simulink model "fault_detection_system_v8"  (R2024a)
settings: Solver=FixedStepDiscrete  StartTime=0.0  StopTime=2  FixedStep=1e-4  RelTol=1e-3
settings Model: Creator=UJJWAL  LastModifiedBy=UJJWAL

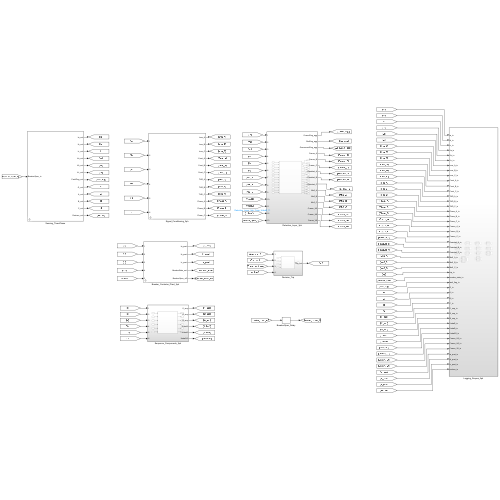
[thumbnail: Simulink's stored preview of the top-level diagram]
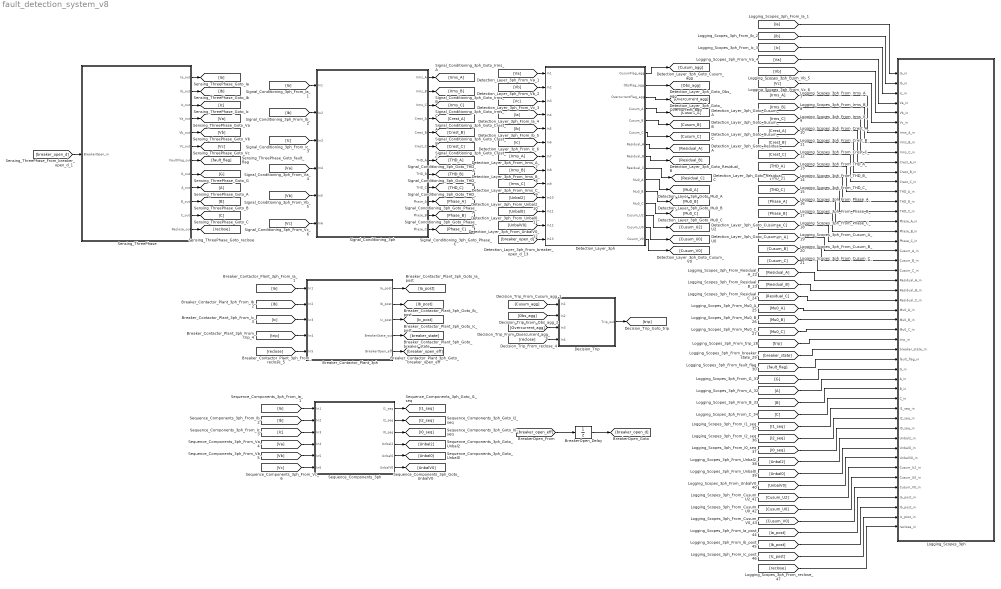
== system fault_detection_system_v8 ==
  BreakerOpen_Delay : UnitDelay  SampleTime=1e-4  HasFrameUpgradeWarning=on
  Breaker_Contactor_Plant_3ph : Subsystem  mask{FeedbackEnable=0, BreakerDelay=0.040000}
      mask prompts: FeedbackEnable "Feedback enable (1 = breaker interrupts the plant, 0 = latch only)"; BreakerDelay "Breaker opening delay after trip command (s)"
  Decision_Trip : Subsystem
  Detection_Layer_3ph : Subsystem
  Logging_Scopes_3ph : Subsystem
  Logging_Scopes_3ph_From_A_32 : From
  Sensing_ThreePhase : Subsystem  mask{FaultG=off, FaultA=on, FaultB=on, FaultC=on, MechanismCode=6, Severity=2750, RampDuration=0, FaultOnsetTime=0.400000, FaultDuration=1.000000, SourceL=0.005, ReclosDelay=0.100000}
      mask prompts: FaultG "Ground involved (G)"; FaultA "Phase A involved"; FaultB "Phase B involved"; FaultC "Phase C involved"; MechanismCode "Mechanism code"; RampDuration "Ramp duration (s)"; FaultOnsetTime "Fault onset time (s)"; FaultDuration "Fault duration (s)"; SourceL "Source inductance (H), 0 = v6 behaviour"; ReclosDelay "Reclose delay after clearance (s)"
  Sensing_ThreePhase_Goto_A : Goto
  Sequence_Components_3ph : Subsystem
  Signal_Conditioning_3ph : Subsystem  mask{NoiseSeed=3028}
      mask prompts: NoiseSeed "Noise seed"
  wires:
  Sensing_ThreePhase/1(Ia_out) -> [Ia]
  Sensing_ThreePhase/2(Ib_out) -> [Ib]
  Sensing_ThreePhase/3(Ic_out) -> [Ic]
  Sensing_ThreePhase/4(Va_out) -> [Va]
  Sensing_ThreePhase/5(Vb_out) -> [Vb]
  Sensing_ThreePhase/6(Vc_out) -> [Vc]
  Sensing_ThreePhase/7(FaultFlag_out) -> [fault_flag]
  Sensing_ThreePhase/8(G_out) -> [G]
  Sensing_ThreePhase/9(A_out) -> Sensing_ThreePhase_Goto_A/1
  Sensing_ThreePhase/10(B_out) -> [B]
  Sensing_ThreePhase/11(C_out) -> [C]
  Sensing_ThreePhase/12(Reclose_out) -> [reclose]
  Signal_Conditioning_3ph/1(Irms_A) -> [Irms_A]
  Signal_Conditioning_3ph/2(Irms_B) -> [Irms_B]
  Signal_Conditioning_3ph/3(Irms_C) -> [Irms_C]
  Signal_Conditioning_3ph/4(Crest_A) -> [Crest_A]
  Signal_Conditioning_3ph/5(Crest_B) -> [Crest_B]
  Signal_Conditioning_3ph/6(Crest_C) -> [Crest_C]
  Signal_Conditioning_3ph/7(THD_A) -> [THD_A]
  Signal_Conditioning_3ph/8(THD_B) -> [THD_B]
  Signal_Conditioning_3ph/9(THD_C) -> [THD_C]
  Signal_Conditioning_3ph/10(Phase_A) -> [Phase_A]
  Signal_Conditioning_3ph/11(Phase_B) -> [Phase_B]
  Signal_Conditioning_3ph/12(Phase_C) -> [Phase_C]
  Sequence_Components_3ph/1(I1_seq) -> [I1_seq]
  Sequence_Components_3ph/2(I2_seq) -> [I2_seq]
  Sequence_Components_3ph/3(I0_seq) -> [I0_seq]
  Sequence_Components_3ph/4(Unbal2) -> [Unbal2]
  Sequence_Components_3ph/5(Unbal0) -> [Unbal0]
  Sequence_Components_3ph/6(UnbalV0) -> [UnbalV0]
  Detection_Layer_3ph/1(CusumFlag_agg) -> [Cusum_agg]
  Detection_Layer_3ph/2(ObsFlag_agg) -> [Obs_agg]
  Detection_Layer_3ph/3(OvercurrentFlag_agg) -> [Overcurrent_agg]
  Detection_Layer_3ph/4(Cusum_A) -> [Cusum_A]
  Detection_Layer_3ph/5(Cusum_B) -> [Cusum_B]
  Detection_Layer_3ph/6(Cusum_C) -> [Cusum_C]
  Detection_Layer_3ph/7(Residual_A) -> [Residual_A]
  Detection_Layer_3ph/8(Residual_B) -> [Residual_B]
  Detection_Layer_3ph/9(Residual_C) -> [Residual_C]
  Detection_Layer_3ph/10(Mu0_A) -> [Mu0_A]
  Detection_Layer_3ph/11(Mu0_B) -> [Mu0_B]
  Detection_Layer_3ph/12(Mu0_C) -> [Mu0_C]
  Detection_Layer_3ph/13(Cusum_U2) -> [Cusum_U2]
  Detection_Layer_3ph/14(Cusum_U0) -> [Cusum_U0]
  Detection_Layer_3ph/15(Cusum_V0) -> [Cusum_V0]
  Decision_Trip/1(Trip_out) -> [trip]
  Breaker_Contactor_Plant_3ph/1(Ia_post) -> [Ia_post]
  Breaker_Contactor_Plant_3ph/2(Ib_post) -> [Ib_post]
  Breaker_Contactor_Plant_3ph/3(Ic_post) -> [Ic_post]
  Breaker_Contactor_Plant_3ph/4(BreakerState_out) -> [breaker_state]
  Breaker_Contactor_Plant_3ph/5(BreakerOpen_eff) -> [breaker_open_eff]
  [breaker_open_d] -> Sensing_ThreePhase/1(BreakerOpen_in)
  [Ia] -> Signal_Conditioning_3ph/1(In1)
  [Ib] -> Signal_Conditioning_3ph/2(In2)
  [Ic] -> Signal_Conditioning_3ph/3(In3)
  [Va] -> Signal_Conditioning_3ph/4(In4)
  [Vb] -> Signal_Conditioning_3ph/5(In5)
  [Vc] -> Signal_Conditioning_3ph/6(In6)
  [Ia] -> Sequence_Components_3ph/1(In1)
  [Ib] -> Sequence_Components_3ph/2(In2)
  [Ic] -> Sequence_Components_3ph/3(In3)
  [Va] -> Sequence_Components_3ph/4(In4)
  [Vb] -> Sequence_Components_3ph/5(In5)
  [Vc] -> Sequence_Components_3ph/6(In6)
  [Va] -> Detection_Layer_3ph/1(In1)
  [Vb] -> Detection_Layer_3ph/2(In2)
  [Vc] -> Detection_Layer_3ph/3(In3)
  [Ia] -> Detection_Layer_3ph/4(In4)
  [Ib] -> Detection_Layer_3ph/5(In5)
  [Ic] -> Detection_Layer_3ph/6(In6)
  [Irms_A] -> Detection_Layer_3ph/7(In7)
  [Irms_B] -> Detection_Layer_3ph/8(In8)
  [Irms_C] -> Detection_Layer_3ph/9(In9)
  [Unbal2] -> Detection_Layer_3ph/10(In10)
  [Unbal0] -> Detection_Layer_3ph/11(In11)
  [UnbalV0] -> Detection_Layer_3ph/12(In12)
  [breaker_open_d] -> Detection_Layer_3ph/13(In13)
  [Cusum_agg] -> Decision_Trip/1(In1)
  [Obs_agg] -> Decision_Trip/2(In2)
  [Overcurrent_agg] -> Decision_Trip/3(In3)
  [reclose] -> Decision_Trip/4(In4)
  [Ia] -> Breaker_Contactor_Plant_3ph/1(In1)
  [Ib] -> Breaker_Contactor_Plant_3ph/2(In2)
  [Ic] -> Breaker_Contactor_Plant_3ph/3(In3)
  [trip] -> Breaker_Contactor_Plant_3ph/4(In4)
  [reclose] -> Breaker_Contactor_Plant_3ph/5(In5)
  [Ia] -> Logging_Scopes_3ph/1(Ia_in)
  [Ib] -> Logging_Scopes_3ph/2(Ib_in)
  [Ic] -> Logging_Scopes_3ph/3(Ic_in)
  [Va] -> Logging_Scopes_3ph/4(Va_in)
  [Vb] -> Logging_Scopes_3ph/5(Vb_in)
  [Vc] -> Logging_Scopes_3ph/6(Vc_in)
  [Irms_A] -> Logging_Scopes_3ph/7(Irms_A_in)
  [Irms_B] -> Logging_Scopes_3ph/8(Irms_B_in)
  [Irms_C] -> Logging_Scopes_3ph/9(Irms_C_in)
  [Crest_A] -> Logging_Scopes_3ph/10(Crest_A_in)
  [Crest_B] -> Logging_Scopes_3ph/11(Crest_B_in)
  [Crest_C] -> Logging_Scopes_3ph/12(Crest_C_in)
  [THD_A] -> Logging_Scopes_3ph/13(THD_A_in)
  [THD_B] -> Logging_Scopes_3ph/14(THD_B_in)
  [THD_C] -> Logging_Scopes_3ph/15(THD_C_in)
  [Phase_A] -> Logging_Scopes_3ph/16(Phase_A_in)
  [Phase_B] -> Logging_Scopes_3ph/17(Phase_B_in)
  [Phase_C] -> Logging_Scopes_3ph/18(Phase_C_in)
  [Cusum_A] -> Logging_Scopes_3ph/19(Cusum_A_in)
  [Cusum_B] -> Logging_Scopes_3ph/20(Cusum_B_in)
  [Cusum_C] -> Logging_Scopes_3ph/21(Cusum_C_in)
  [Residual_A] -> Logging_Scopes_3ph/22(Residual_A_in)
  [Residual_B] -> Logging_Scopes_3ph/23(Residual_B_in)
  [Residual_C] -> Logging_Scopes_3ph/24(Residual_C_in)
  [Mu0_A] -> Logging_Scopes_3ph/25(Mu0_A_in)
  [Mu0_B] -> Logging_Scopes_3ph/26(Mu0_B_in)
  [Mu0_C] -> Logging_Scopes_3ph/27(Mu0_C_in)
  [trip] -> Logging_Scopes_3ph/28(trip_in)
  [breaker_state] -> Logging_Scopes_3ph/29(breaker_state_in)
  [fault_flag] -> Logging_Scopes_3ph/30(fault_flag_in)
  [G] -> Logging_Scopes_3ph/31(G_in)
  Logging_Scopes_3ph_From_A_32/1 -> Logging_Scopes_3ph/32(A_in)
  [B] -> Logging_Scopes_3ph/33(B_in)
  [C] -> Logging_Scopes_3ph/34(C_in)
  [I1_seq] -> Logging_Scopes_3ph/35(I1_seq_in)
  [I2_seq] -> Logging_Scopes_3ph/36(I2_seq_in)
  [I0_seq] -> Logging_Scopes_3ph/37(I0_seq_in)
  [Unbal2] -> Logging_Scopes_3ph/38(Unbal2_in)
  [Unbal0] -> Logging_Scopes_3ph/39(Unbal0_in)
  [UnbalV0] -> Logging_Scopes_3ph/40(UnbalV0_in)
  [Cusum_U2] -> Logging_Scopes_3ph/41(Cusum_U2_in)
  [Cusum_U0] -> Logging_Scopes_3ph/42(Cusum_U0_in)
  [Cusum_V0] -> Logging_Scopes_3ph/43(Cusum_V0_in)
  [Ia_post] -> Logging_Scopes_3ph/44(Ia_post_in)
  [Ib_post] -> Logging_Scopes_3ph/45(Ib_post_in)
  [Ic_post] -> Logging_Scopes_3ph/46(Ic_post_in)
  [reclose] -> Logging_Scopes_3ph/47(reclose_in)
  [breaker_open_eff] -> BreakerOpen_Delay/1
  BreakerOpen_Delay/1 -> [breaker_open_d]

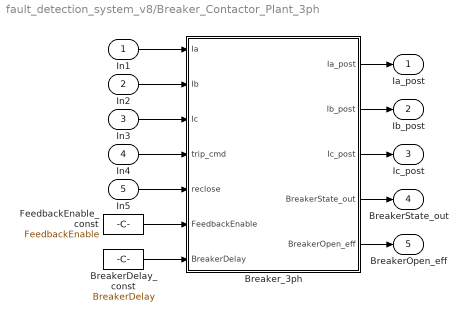
== system fault_detection_system_v8/Breaker_Contactor_Plant_3ph ==
  In1 : Inport
  In2 : Inport  Port=2
  In3 : Inport  Port=3
  In4 : Inport  Port=4
  In5 : Inport  Port=5
  BreakerDelay_const : Constant  Value=BreakerDelay
  Breaker_3ph : MATLAB Function  TreatAsAtomicUnit=on
  FeedbackEnable_const : Constant  Value=FeedbackEnable
  Ia_post : Outport
  Ib_post : Outport  Port=2
  Ic_post : Outport  Port=3
  BreakerState_out : Outport  Port=4
  BreakerOpen_eff : Outport  Port=5
  wires:
  Breaker_3ph/1(Ia_post) -> Ia_post/1
  Breaker_3ph/2(Ib_post) -> Ib_post/1
  Breaker_3ph/3(Ic_post) -> Ic_post/1
  Breaker_3ph/4(BreakerState_out) -> BreakerState_out/1
  Breaker_3ph/5(BreakerOpen_eff) -> BreakerOpen_eff/1
  In1/1 -> Breaker_3ph/1(Ia)
  In2/1 -> Breaker_3ph/2(Ib)
  In3/1 -> Breaker_3ph/3(Ic)
  In4/1 -> Breaker_3ph/4(trip_cmd)
  In5/1 -> Breaker_3ph/5(reclose)
  FeedbackEnable_const/1 -> Breaker_3ph/6(FeedbackEnable)
  BreakerDelay_const/1 -> Breaker_3ph/7(BreakerDelay)

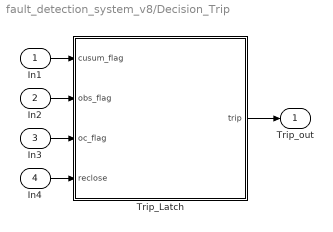
== system fault_detection_system_v8/Decision_Trip ==
  In1 : Inport
  In2 : Inport  Port=2
  In3 : Inport  Port=3
  In4 : Inport  Port=4
  Trip_Latch : MATLAB Function  TreatAsAtomicUnit=on
  Trip_out : Outport
  wires:
  In1/1 -> Trip_Latch/1(cusum_flag)
  In2/1 -> Trip_Latch/2(obs_flag)
  In3/1 -> Trip_Latch/3(oc_flag)
  In4/1 -> Trip_Latch/4(reclose)
  Trip_Latch/1(trip) -> Trip_out/1

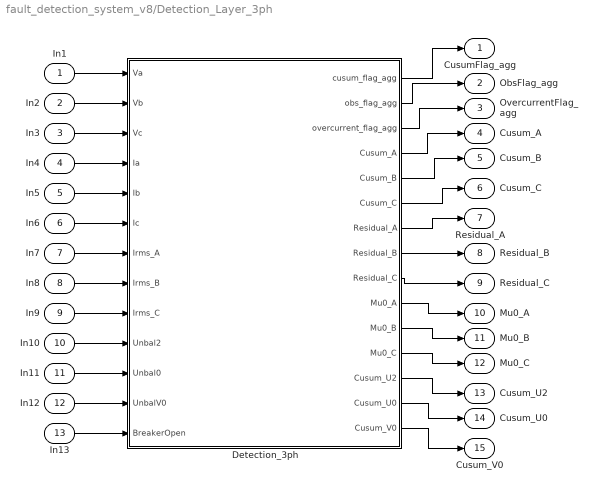
== system fault_detection_system_v8/Detection_Layer_3ph ==
  In1 : Inport
  In2 : Inport  Port=2
  In3 : Inport  Port=3
  In4 : Inport  Port=4
  In5 : Inport  Port=5
  In6 : Inport  Port=6
  In7 : Inport  Port=7
  In8 : Inport  Port=8
  In9 : Inport  Port=9
  In10 : Inport  Port=10
  In11 : Inport  Port=11
  In12 : Inport  Port=12
  In13 : Inport  Port=13
  Detection_3ph : MATLAB Function  TreatAsAtomicUnit=on
  CusumFlag_agg : Outport
  ObsFlag_agg : Outport  Port=2
  OvercurrentFlag_agg : Outport  Port=3
  Cusum_A : Outport  Port=4
  Cusum_B : Outport  Port=5
  Cusum_C : Outport  Port=6
  Residual_A : Outport  Port=7
  Residual_B : Outport  Port=8
  Residual_C : Outport  Port=9
  Mu0_A : Outport  Port=10
  Mu0_B : Outport  Port=11
  Mu0_C : Outport  Port=12
  Cusum_U2 : Outport  Port=13
  Cusum_U0 : Outport  Port=14
  Cusum_V0 : Outport  Port=15
  wires:
  Detection_3ph/1(cusum_flag_agg) -> CusumFlag_agg/1
  Detection_3ph/2(obs_flag_agg) -> ObsFlag_agg/1
  Detection_3ph/3(overcurrent_flag_agg) -> OvercurrentFlag_agg/1
  Detection_3ph/4(Cusum_A) -> Cusum_A/1
  Detection_3ph/5(Cusum_B) -> Cusum_B/1
  Detection_3ph/6(Cusum_C) -> Cusum_C/1
  Detection_3ph/7(Residual_A) -> Residual_A/1
  Detection_3ph/8(Residual_B) -> Residual_B/1
  Detection_3ph/9(Residual_C) -> Residual_C/1
  Detection_3ph/10(Mu0_A) -> Mu0_A/1
  Detection_3ph/11(Mu0_B) -> Mu0_B/1
  Detection_3ph/12(Mu0_C) -> Mu0_C/1
  Detection_3ph/13(Cusum_U2) -> Cusum_U2/1
  Detection_3ph/14(Cusum_U0) -> Cusum_U0/1
  Detection_3ph/15(Cusum_V0) -> Cusum_V0/1
  In1/1 -> Detection_3ph/1(Va)
  In2/1 -> Detection_3ph/2(Vb)
  In3/1 -> Detection_3ph/3(Vc)
  In4/1 -> Detection_3ph/4(Ia)
  In5/1 -> Detection_3ph/5(Ib)
  In6/1 -> Detection_3ph/6(Ic)
  In7/1 -> Detection_3ph/7(Irms_A)
  In8/1 -> Detection_3ph/8(Irms_B)
  In9/1 -> Detection_3ph/9(Irms_C)
  In10/1 -> Detection_3ph/10(Unbal2)
  In11/1 -> Detection_3ph/11(Unbal0)
  In12/1 -> Detection_3ph/12(UnbalV0)
  In13/1 -> Detection_3ph/13(BreakerOpen)

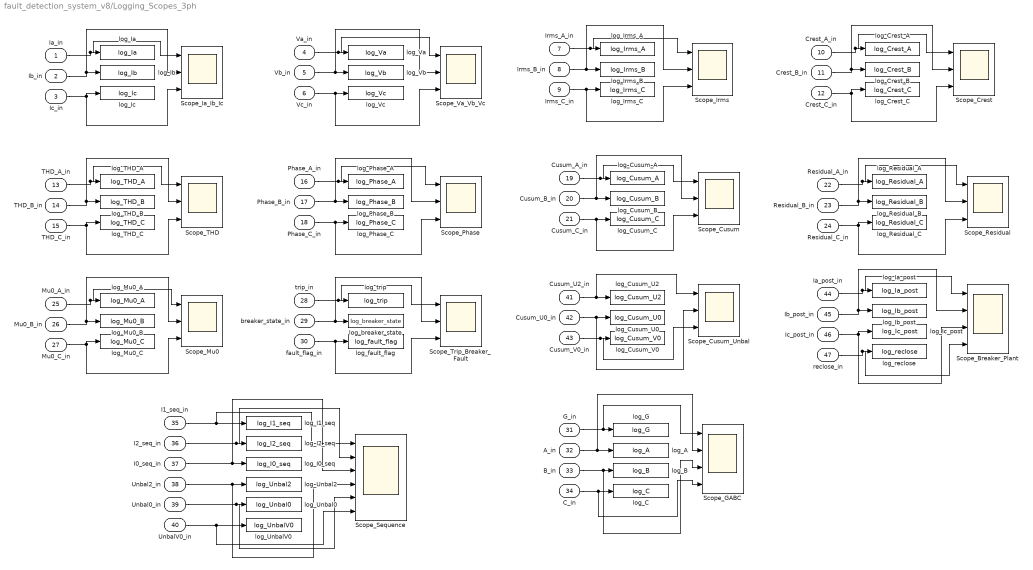
== system fault_detection_system_v8/Logging_Scopes_3ph ==
  Ia_in : Inport
  Ib_in : Inport  Port=2
  Ic_in : Inport  Port=3
  Va_in : Inport  Port=4
  Vb_in : Inport  Port=5
  Vc_in : Inport  Port=6
  Irms_A_in : Inport  Port=7
  Irms_B_in : Inport  Port=8
  Irms_C_in : Inport  Port=9
  Crest_A_in : Inport  Port=10
  Crest_B_in : Inport  Port=11
  Crest_C_in : Inport  Port=12
  THD_A_in : Inport  Port=13
  THD_B_in : Inport  Port=14
  THD_C_in : Inport  Port=15
  Phase_A_in : Inport  Port=16
  Phase_B_in : Inport  Port=17
  Phase_C_in : Inport  Port=18
  Cusum_A_in : Inport  Port=19
  Cusum_B_in : Inport  Port=20
  Cusum_C_in : Inport  Port=21
  Residual_A_in : Inport  Port=22
  Residual_B_in : Inport  Port=23
  Residual_C_in : Inport  Port=24
  Mu0_A_in : Inport  Port=25
  Mu0_B_in : Inport  Port=26
  Mu0_C_in : Inport  Port=27
  trip_in : Inport  Port=28
  breaker_state_in : Inport  Port=29
  fault_flag_in : Inport  Port=30
  G_in : Inport  Port=31
  A_in : Inport  Port=32
  B_in : Inport  Port=33
  C_in : Inport  Port=34
  I1_seq_in : Inport  Port=35
  I2_seq_in : Inport  Port=36
  I0_seq_in : Inport  Port=37
  Unbal2_in : Inport  Port=38
  Unbal0_in : Inport  Port=39
  UnbalV0_in : Inport  Port=40
  Cusum_U2_in : Inport  Port=41
  Cusum_U0_in : Inport  Port=42
  Cusum_V0_in : Inport  Port=43
  Ia_post_in : Inport  Port=44
  Ib_post_in : Inport  Port=45
  Ic_post_in : Inport  Port=46
  reclose_in : Inport  Port=47
  Scope_Breaker_Plant : Scope  NumInputPorts=4
  Scope_Crest : Scope  NumInputPorts=3
  Scope_Cusum : Scope  NumInputPorts=3
  Scope_Cusum_Unbal : Scope  NumInputPorts=3
  Scope_GABC : Scope  NumInputPorts=4
  Scope_Ia_Ib_Ic : Scope  NumInputPorts=3
  Scope_Irms : Scope  NumInputPorts=3
  Scope_Mu0 : Scope  NumInputPorts=3
  Scope_Phase : Scope  NumInputPorts=3
  Scope_Residual : Scope  NumInputPorts=3
  Scope_Sequence : Scope  NumInputPorts=6
  Scope_THD : Scope  NumInputPorts=3
  Scope_Trip_Breaker_Fault : Scope  NumInputPorts=3
  Scope_Va_Vb_Vc : Scope  NumInputPorts=3
  log_A : ToWorkspace  VariableName=log_A  SaveFormat=Timeseries  SampleTime=-1
  log_B : ToWorkspace  VariableName=log_B  SaveFormat=Timeseries  SampleTime=-1
  log_C : ToWorkspace  VariableName=log_C  SaveFormat=Timeseries  SampleTime=-1
  log_Crest_A : ToWorkspace  VariableName=log_Crest_A  SaveFormat=Timeseries  SampleTime=-1
  log_Crest_B : ToWorkspace  VariableName=log_Crest_B  SaveFormat=Timeseries  SampleTime=-1
  log_Crest_C : ToWorkspace  VariableName=log_Crest_C  SaveFormat=Timeseries  SampleTime=-1
  log_Cusum_A : ToWorkspace  VariableName=log_Cusum_A  SaveFormat=Timeseries  SampleTime=-1
  log_Cusum_B : ToWorkspace  VariableName=log_Cusum_B  SaveFormat=Timeseries  SampleTime=-1
  log_Cusum_C : ToWorkspace  VariableName=log_Cusum_C  SaveFormat=Timeseries  SampleTime=-1
  log_Cusum_U0 : ToWorkspace  VariableName=log_Cusum_U0  SaveFormat=Timeseries  SampleTime=-1
  log_Cusum_U2 : ToWorkspace  VariableName=log_Cusum_U2  SaveFormat=Timeseries  SampleTime=-1
  log_Cusum_V0 : ToWorkspace  VariableName=log_Cusum_V0  SaveFormat=Timeseries  SampleTime=-1
  log_G : ToWorkspace  VariableName=log_G  SaveFormat=Timeseries  SampleTime=-1
  log_I0_seq : ToWorkspace  VariableName=log_I0_seq  SaveFormat=Timeseries  SampleTime=-1
  log_I1_seq : ToWorkspace  VariableName=log_I1_seq  SaveFormat=Timeseries  SampleTime=-1
  log_I2_seq : ToWorkspace  VariableName=log_I2_seq  SaveFormat=Timeseries  SampleTime=-1
  log_Ia : ToWorkspace  VariableName=log_Ia  SaveFormat=Timeseries  SampleTime=-1
  log_Ia_post : ToWorkspace  VariableName=log_Ia_post  SaveFormat=Timeseries  SampleTime=-1
  log_Ib : ToWorkspace  VariableName=log_Ib  SaveFormat=Timeseries  SampleTime=-1
  log_Ib_post : ToWorkspace  VariableName=log_Ib_post  SaveFormat=Timeseries  SampleTime=-1
  log_Ic : ToWorkspace  VariableName=log_Ic  SaveFormat=Timeseries  SampleTime=-1
  log_Ic_post : ToWorkspace  VariableName=log_Ic_post  SaveFormat=Timeseries  SampleTime=-1
  log_Irms_A : ToWorkspace  VariableName=log_Irms_A  SaveFormat=Timeseries  SampleTime=-1
  log_Irms_B : ToWorkspace  VariableName=log_Irms_B  SaveFormat=Timeseries  SampleTime=-1
  log_Irms_C : ToWorkspace  VariableName=log_Irms_C  SaveFormat=Timeseries  SampleTime=-1
  log_Mu0_A : ToWorkspace  VariableName=log_Mu0_A  SaveFormat=Timeseries  SampleTime=-1
  log_Mu0_B : ToWorkspace  VariableName=log_Mu0_B  SaveFormat=Timeseries  SampleTime=-1
  log_Mu0_C : ToWorkspace  VariableName=log_Mu0_C  SaveFormat=Timeseries  SampleTime=-1
  log_Phase_A : ToWorkspace  VariableName=log_Phase_A  SaveFormat=Timeseries  SampleTime=-1
  log_Phase_B : ToWorkspace  VariableName=log_Phase_B  SaveFormat=Timeseries  SampleTime=-1
  log_Phase_C : ToWorkspace  VariableName=log_Phase_C  SaveFormat=Timeseries  SampleTime=-1
  log_Residual_A : ToWorkspace  VariableName=log_Residual_A  SaveFormat=Timeseries  SampleTime=-1
  log_Residual_B : ToWorkspace  VariableName=log_Residual_B  SaveFormat=Timeseries  SampleTime=-1
  log_Residual_C : ToWorkspace  VariableName=log_Residual_C  SaveFormat=Timeseries  SampleTime=-1
  log_THD_A : ToWorkspace  VariableName=log_THD_A  SaveFormat=Timeseries  SampleTime=-1
  log_THD_B : ToWorkspace  VariableName=log_THD_B  SaveFormat=Timeseries  SampleTime=-1
  log_THD_C : ToWorkspace  VariableName=log_THD_C  SaveFormat=Timeseries  SampleTime=-1
  log_Unbal0 : ToWorkspace  VariableName=log_Unbal0  SaveFormat=Timeseries  SampleTime=-1
  log_Unbal2 : ToWorkspace  VariableName=log_Unbal2  SaveFormat=Timeseries  SampleTime=-1
  log_UnbalV0 : ToWorkspace  VariableName=log_UnbalV0  SaveFormat=Timeseries  SampleTime=-1
  log_Va : ToWorkspace  VariableName=log_Va  SaveFormat=Timeseries  SampleTime=-1
  log_Vb : ToWorkspace  VariableName=log_Vb  SaveFormat=Timeseries  SampleTime=-1
  log_Vc : ToWorkspace  VariableName=log_Vc  SaveFormat=Timeseries  SampleTime=-1
  log_breaker_state : ToWorkspace  VariableName=log_breaker_state  SaveFormat=Timeseries  SampleTime=-1
  log_fault_flag : ToWorkspace  VariableName=log_fault_flag  SaveFormat=Timeseries  SampleTime=-1
  log_reclose : ToWorkspace  VariableName=log_reclose  SaveFormat=Timeseries  SampleTime=-1
  log_trip : ToWorkspace  VariableName=log_trip  SaveFormat=Timeseries  SampleTime=-1
  wires:
  Ia_in/1 -> log_Ia/1, Scope_Ia_Ib_Ic/1
  Ib_in/1 -> log_Ib/1, Scope_Ia_Ib_Ic/2
  Ic_in/1 -> log_Ic/1, Scope_Ia_Ib_Ic/3
  Va_in/1 -> log_Va/1, Scope_Va_Vb_Vc/1
  Vb_in/1 -> log_Vb/1, Scope_Va_Vb_Vc/2
  Vc_in/1 -> log_Vc/1, Scope_Va_Vb_Vc/3
  Irms_A_in/1 -> log_Irms_A/1, Scope_Irms/1
  Irms_B_in/1 -> log_Irms_B/1, Scope_Irms/2
  Irms_C_in/1 -> log_Irms_C/1, Scope_Irms/3
  Crest_A_in/1 -> log_Crest_A/1, Scope_Crest/1
  Crest_B_in/1 -> log_Crest_B/1, Scope_Crest/2
  Crest_C_in/1 -> log_Crest_C/1, Scope_Crest/3
  THD_A_in/1 -> log_THD_A/1, Scope_THD/1
  THD_B_in/1 -> log_THD_B/1, Scope_THD/2
  THD_C_in/1 -> log_THD_C/1, Scope_THD/3
  Phase_A_in/1 -> log_Phase_A/1, Scope_Phase/1
  Phase_B_in/1 -> log_Phase_B/1, Scope_Phase/2
  Phase_C_in/1 -> log_Phase_C/1, Scope_Phase/3
  Cusum_A_in/1 -> log_Cusum_A/1, Scope_Cusum/1
  Cusum_B_in/1 -> log_Cusum_B/1, Scope_Cusum/2
  Cusum_C_in/1 -> log_Cusum_C/1, Scope_Cusum/3
  Residual_A_in/1 -> log_Residual_A/1, Scope_Residual/1
  Residual_B_in/1 -> log_Residual_B/1, Scope_Residual/2
  Residual_C_in/1 -> log_Residual_C/1, Scope_Residual/3
  Mu0_A_in/1 -> log_Mu0_A/1, Scope_Mu0/1
  Mu0_B_in/1 -> log_Mu0_B/1, Scope_Mu0/2
  Mu0_C_in/1 -> log_Mu0_C/1, Scope_Mu0/3
  trip_in/1 -> log_trip/1, Scope_Trip_Breaker_Fault/1
  breaker_state_in/1 -> log_breaker_state/1, Scope_Trip_Breaker_Fault/2
  fault_flag_in/1 -> log_fault_flag/1, Scope_Trip_Breaker_Fault/3
  G_in/1 -> log_G/1, Scope_GABC/1
  A_in/1 -> log_A/1, Scope_GABC/2
  B_in/1 -> log_B/1, Scope_GABC/3
  C_in/1 -> log_C/1, Scope_GABC/4
  I1_seq_in/1 -> log_I1_seq/1, Scope_Sequence/1
  I2_seq_in/1 -> log_I2_seq/1, Scope_Sequence/2
  I0_seq_in/1 -> log_I0_seq/1, Scope_Sequence/3
  Unbal2_in/1 -> log_Unbal2/1, Scope_Sequence/4
  Unbal0_in/1 -> log_Unbal0/1, Scope_Sequence/5
  UnbalV0_in/1 -> log_UnbalV0/1, Scope_Sequence/6
  Cusum_U2_in/1 -> log_Cusum_U2/1, Scope_Cusum_Unbal/1
  Cusum_U0_in/1 -> log_Cusum_U0/1, Scope_Cusum_Unbal/2
  Cusum_V0_in/1 -> log_Cusum_V0/1, Scope_Cusum_Unbal/3
  Ia_post_in/1 -> log_Ia_post/1, Scope_Breaker_Plant/1
  Ib_post_in/1 -> log_Ib_post/1, Scope_Breaker_Plant/2
  Ic_post_in/1 -> log_Ic_post/1, Scope_Breaker_Plant/3
  reclose_in/1 -> log_reclose/1, Scope_Breaker_Plant/4

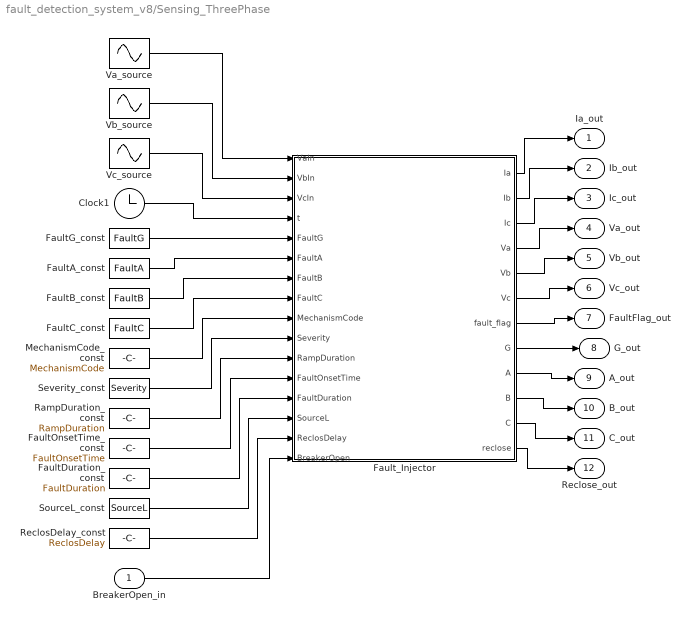
== system fault_detection_system_v8/Sensing_ThreePhase ==
  BreakerOpen_in : Inport
  Clock1 : Clock
  FaultA_const : Constant  Value=FaultA
  FaultB_const : Constant  Value=FaultB
  FaultC_const : Constant  Value=FaultC
  FaultDuration_const : Constant  Value=FaultDuration
  FaultG_const : Constant  Value=FaultG
  FaultOnsetTime_const : Constant  Value=FaultOnsetTime
  Fault_Injector : MATLAB Function  TreatAsAtomicUnit=on
  MechanismCode_const : Constant  Value=MechanismCode
  RampDuration_const : Constant  Value=RampDuration
  ReclosDelay_const : Constant  Value=ReclosDelay
  Severity_const : Constant  Value=Severity
  SourceL_const : Constant  Value=SourceL
  Va_source : Sin  Amplitude=325  Frequency=314.159  SampleTime=0
  Vb_source : Sin  Amplitude=325  Frequency=314.159  Phase=-2.0944  SampleTime=0
  Vc_source : Sin  Amplitude=325  Frequency=314.159  Phase=2.0944  SampleTime=0
  Ia_out : Outport
  Ib_out : Outport  Port=2
  Ic_out : Outport  Port=3
  Va_out : Outport  Port=4
  Vb_out : Outport  Port=5
  Vc_out : Outport  Port=6
  FaultFlag_out : Outport  Port=7
  G_out : Outport  Port=8
  A_out : Outport  Port=9
  B_out : Outport  Port=10
  C_out : Outport  Port=11
  Reclose_out : Outport  Port=12
  wires:
  FaultG_const/1 -> Fault_Injector/5(FaultG)
  FaultA_const/1 -> Fault_Injector/6(FaultA)
  FaultB_const/1 -> Fault_Injector/7(FaultB)
  FaultC_const/1 -> Fault_Injector/8(FaultC)
  MechanismCode_const/1 -> Fault_Injector/9(MechanismCode)
  Severity_const/1 -> Fault_Injector/10(Severity)
  RampDuration_const/1 -> Fault_Injector/11(RampDuration)
  FaultOnsetTime_const/1 -> Fault_Injector/12(FaultOnsetTime)
  FaultDuration_const/1 -> Fault_Injector/13(FaultDuration)
  SourceL_const/1 -> Fault_Injector/14(SourceL)
  ReclosDelay_const/1 -> Fault_Injector/15(ReclosDelay)
  BreakerOpen_in/1 -> Fault_Injector/16(BreakerOpen)
  Va_source/1 -> Fault_Injector/1(VaIn)
  Vb_source/1 -> Fault_Injector/2(VbIn)
  Vc_source/1 -> Fault_Injector/3(VcIn)
  Clock1/1 -> Fault_Injector/4(t)
  Fault_Injector/1(Ia) -> Ia_out/1
  Fault_Injector/2(Ib) -> Ib_out/1
  Fault_Injector/3(Ic) -> Ic_out/1
  Fault_Injector/4(Va) -> Va_out/1
  Fault_Injector/5(Vb) -> Vb_out/1
  Fault_Injector/6(Vc) -> Vc_out/1
  Fault_Injector/7(fault_flag) -> FaultFlag_out/1
  Fault_Injector/8(G) -> G_out/1
  Fault_Injector/9(A) -> A_out/1
  Fault_Injector/10(B) -> B_out/1
  Fault_Injector/11(C) -> C_out/1
  Fault_Injector/12(reclose) -> Reclose_out/1

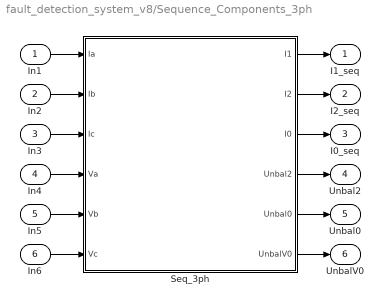
== system fault_detection_system_v8/Sequence_Components_3ph ==
  In1 : Inport
  In2 : Inport  Port=2
  In3 : Inport  Port=3
  In4 : Inport  Port=4
  In5 : Inport  Port=5
  In6 : Inport  Port=6
  Seq_3ph : MATLAB Function  TreatAsAtomicUnit=on
  I1_seq : Outport
  I2_seq : Outport  Port=2
  I0_seq : Outport  Port=3
  Unbal2 : Outport  Port=4
  Unbal0 : Outport  Port=5
  UnbalV0 : Outport  Port=6
  wires:
  Seq_3ph/1(I1) -> I1_seq/1
  Seq_3ph/2(I2) -> I2_seq/1
  Seq_3ph/3(I0) -> I0_seq/1
  Seq_3ph/4(Unbal2) -> Unbal2/1
  Seq_3ph/5(Unbal0) -> Unbal0/1
  Seq_3ph/6(UnbalV0) -> UnbalV0/1
  In1/1 -> Seq_3ph/1(Ia)
  In2/1 -> Seq_3ph/2(Ib)
  In3/1 -> Seq_3ph/3(Ic)
  In4/1 -> Seq_3ph/4(Va)
  In5/1 -> Seq_3ph/5(Vb)
  In6/1 -> Seq_3ph/6(Vc)

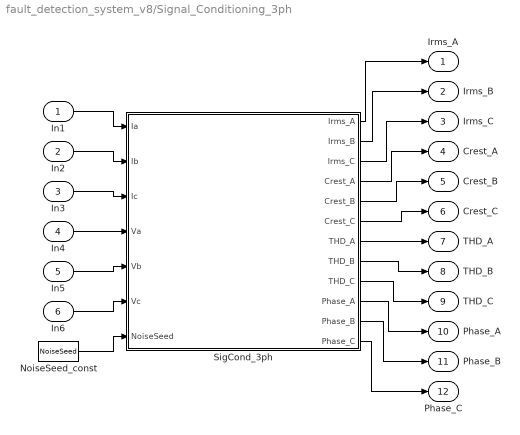
== system fault_detection_system_v8/Signal_Conditioning_3ph ==
  In1 : Inport
  In2 : Inport  Port=2
  In3 : Inport  Port=3
  In4 : Inport  Port=4
  In5 : Inport  Port=5
  In6 : Inport  Port=6
  NoiseSeed_const : Constant  Value=NoiseSeed
  SigCond_3ph : MATLAB Function  TreatAsAtomicUnit=on
  Irms_A : Outport
  Irms_B : Outport  Port=2
  Irms_C : Outport  Port=3
  Crest_A : Outport  Port=4
  Crest_B : Outport  Port=5
  Crest_C : Outport  Port=6
  THD_A : Outport  Port=7
  THD_B : Outport  Port=8
  THD_C : Outport  Port=9
  Phase_A : Outport  Port=10
  Phase_B : Outport  Port=11
  Phase_C : Outport  Port=12
  wires:
  SigCond_3ph/1(Irms_A) -> Irms_A/1
  SigCond_3ph/2(Irms_B) -> Irms_B/1
  SigCond_3ph/3(Irms_C) -> Irms_C/1
  SigCond_3ph/4(Crest_A) -> Crest_A/1
  SigCond_3ph/5(Crest_B) -> Crest_B/1
  SigCond_3ph/6(Crest_C) -> Crest_C/1
  SigCond_3ph/7(THD_A) -> THD_A/1
  SigCond_3ph/8(THD_B) -> THD_B/1
  SigCond_3ph/9(THD_C) -> THD_C/1
  SigCond_3ph/10(Phase_A) -> Phase_A/1
  SigCond_3ph/11(Phase_B) -> Phase_B/1
  SigCond_3ph/12(Phase_C) -> Phase_C/1
  In1/1 -> SigCond_3ph/1(Ia)
  In2/1 -> SigCond_3ph/2(Ib)
  In3/1 -> SigCond_3ph/3(Ic)
  In4/1 -> SigCond_3ph/4(Va)
  In5/1 -> SigCond_3ph/5(Vb)
  In6/1 -> SigCond_3ph/6(Vc)
  NoiseSeed_const/1 -> SigCond_3ph/7(NoiseSeed)

== matlab function fault_detection_system_v8/Detection_Layer_3ph/Detection_3ph ==
  data: Va input; cusum_flag_agg output; Vb input; Vc input; Ia input; Ib input; Ic input; Irms_A input; Irms_B input; Irms_C input; Unbal2 input; Unbal0 input; UnbalV0 input; BreakerOpen input; obs_flag_agg output; overcurrent_flag_agg output; Cusum_A output; Cusum_B output; Cusum_C output; Residual_A output; Residual_B output; Residual_C output; Mu0_A output; Mu0_B output; Mu0_C output; Cusum_U2 output; Cusum_U0 output; Cusum_V0 output
function [cusum_flag_agg,obs_flag_agg,overcurrent_flag_agg,Cusum_A,Cusum_B,Cusum_C,Residual_A,Residual_B,Residual_C,Mu0_A,Mu0_B,Mu0_C,Cusum_U2,Cusum_U0,Cusum_V0] = detection_3ph(Va,Vb,Vc,Ia,Ib,Ic,Irms_A,Irms_B,Irms_C,Unbal2,Unbal0,UnbalV0,BreakerOpen)
    persistent mu0 var0 g_pos g_neg initialized sampleCount WARMUP_SAMPLES SETTLE_SAMPLES settleCount blank
    if isempty(initialized)
        mu0 = zeros(6,1); var0 = [0.01; 0.01; 0.01; 1e-6; 1e-6; 1e-6];
        g_pos = zeros(6,1); g_neg = zeros(6,1); initialized = true;
        sampleCount = 0; WARMUP_SAMPLES = 500; SETTLE_SAMPLES = 400; settleCount = 0; blank = 0;
    end
    sampleCount = sampleCount + 1;
    HOLD_SAMPLES = 500;   % 50 ms hold after the breaker closes again (lets the 200-sample windows refill)
    CUSUM_CAP = 10;       % anti-windup: CUSUM statistic is capped at CUSUM_CAP * H_THRESH
    if BreakerOpen > 0.5
        blank = HOLD_SAMPLES;
    elseif blank > 0
        blank = blank - 1;
    end
    hold_det = blank > 0;
    % 6 Channels: Irms A, B, C | Unbal2 | Unbal0 | UnbalV0 (the last three are dimensionless)
    x = [Irms_A; Irms_B; Irms_C; Unbal2; Unbal0; UnbalV0];
    err = x - mu0; residual = abs(err);
    % Minimum noise floor: 0.05 A for Irms, 0.005 (0.5 percent of the healthy reference) for the unbalance channels
    NOISE_FLOOR = [0.05; 0.05; 0.05; 0.005; 0.005; 0.005];
    std0 = max(sqrt(var0), NOISE_FLOOR);
    k = 1.0 * std0; H_THRESH = 10 * std0; OVERCURRENT_THRESH = mu0 + 15 * std0;
    if sampleCount <= WARMUP_SAMPLES
        if sampleCount > SETTLE_SAMPLES
            settleCount = settleCount + 1; delta = x - mu0;
            mu0 = mu0 + delta / settleCount; var0 = var0 + (delta .* (x - mu0) - var0) / settleCount;
        end
        g_pos = zeros(6,1); g_neg = zeros(6,1); cusum_stat = zeros(6,1);
        cusum_flag_ph = false(6,1); obs_flag_ph = false(6,1); overcurrent_flag_ph = false(6,1);
    elseif hold_det
        % Breaker open (or just closed): statistics held at zero, no flags, mu0 / var0 frozen
        g_pos = zeros(6,1); g_neg = zeros(6,1); cusum_stat = zeros(6,1);
        cusum_flag_ph = false(6,1); obs_flag_ph = false(6,1); overcurrent_flag_ph = false(6,1);
    else
        g_pos = min(max(0, g_pos + err - k), CUSUM_CAP * H_THRESH); g_neg = min(max(0, g_neg - err - k), CUSUM_CAP * H_THRESH);
        cusum_stat = max(g_pos, g_neg); cusum_flag_ph = cusum_stat > H_THRESH;
        obs_flag_ph = residual > 5 * std0; overcurrent_flag_ph = x > OVERCURRENT_THRESH;
        overcurrent_flag_ph(4:6) = false;   % Upper limit disabled for the unbalance channels
        normal_mask = ~(cusum_flag_ph | obs_flag_ph | overcurrent_flag_ph);
        delta_norm = x(normal_mask) - mu0(normal_mask);
        mu0(normal_mask) = 0.999 * mu0(normal_mask) + 0.001 * x(normal_mask);
        var0(normal_mask) = 0.999 * var0(normal_mask) + 0.001 * (delta_norm.^2);
    end
    cusum_flag_agg = any(cusum_flag_ph); obs_flag_agg = any(obs_flag_ph); overcurrent_flag_agg = any(overcurrent_flag_ph);
    Cusum_A = cusum_stat(1); Cusum_B = cusum_stat(2); Cusum_C = cusum_stat(3);
    Residual_A = residual(1); Residual_B = residual(2); Residual_C = residual(3);
    Mu0_A = mu0(1); Mu0_B = mu0(2); Mu0_C = mu0(3);
    Cusum_U2 = cusum_stat(4); Cusum_U0 = cusum_stat(5); Cusum_V0 = cusum_stat(6);
end

== matlab function fault_detection_system_v8/Decision_Trip/Trip_Latch ==
  data: cusum_flag input; trip output; obs_flag input; oc_flag input; reclose input
function trip = trip_latch(cusum_flag, obs_flag, oc_flag, reclose)
%#codegen
persistent latch cnt
if isempty(latch), latch = false; cnt = 0; end
CONFIRM_SAMPLES = 50;   % trip confirmation: a detector flag must stay high this many samples (50 x 0.1 ms = 5 ms, a quarter cycle)
anyFlag = (double(cusum_flag) > 0.5) || (double(obs_flag) > 0.5) || (double(oc_flag) > 0.5);
if anyFlag, cnt = cnt + 1; else, cnt = 0; end
if double(reclose) > 0.5
    latch = false; cnt = 0;
elseif cnt >= CONFIRM_SAMPLES
    latch = true;
end
trip = double(latch);
end

== matlab function fault_detection_system_v8/Breaker_Contactor_Plant_3ph/Breaker_3ph ==
  data: Ia input; Ia_post output; Ib input; Ic input; trip_cmd input; reclose input; FeedbackEnable input; BreakerDelay input; Ib_post output; Ic_post output; BreakerState_out output; BreakerOpen_eff output
function [Ia_post,Ib_post,Ic_post,BreakerState_out,BreakerOpen_eff] = breaker_3ph(Ia,Ib,Ic,trip_cmd,reclose,FeedbackEnable,BreakerDelay)
%#codegen
persistent state tcnt
if isempty(state), state = 0; tcnt = 0; end
Ts = 1e-4;
delaySamples = round(BreakerDelay / Ts);
if reclose > 0.5
    state = 0; tcnt = 0;
else
    if trip_cmd > 0.5, tcnt = tcnt + 1; end
    if trip_cmd > 0.5 && tcnt > delaySamples, state = 1; end
end
Ia_post = Ia * (1 - state); Ib_post = Ib * (1 - state); Ic_post = Ic * (1 - state);
BreakerState_out = state;
% only this effective state is fed back to the plant and the detector; FeedbackEnable = 0 keeps the v6 behaviour
BreakerOpen_eff = state * double(FeedbackEnable > 0.5);
end

== matlab function fault_detection_system_v8/Signal_Conditioning_3ph/SigCond_3ph ==
  data: Ia input; Irms_A output; Ib input; Ic input; Va input; Vb input; Vc input; NoiseSeed input; Irms_B output; Irms_C output; Crest_A output; Crest_B output; Crest_C output; THD_A output; THD_B output; THD_C output; Phase_A output; Phase_B output; Phase_C output
function [Irms_A,Irms_B,Irms_C,Crest_A,Crest_B,Crest_C,THD_A,THD_B,THD_C,Phase_A,Phase_B,Phase_C] = sigcond_3ph(Ia,Ib,Ic,Va,Vb,Vc,NoiseSeed)
%#codegen
persistent bufI bufV idx N rngState
if isempty(idx)
    N = 200; bufI = zeros(3,N); bufV = zeros(3,N); idx = 1;
    s0 = mod(double(NoiseSeed) * 2654435761 + 12345, 4294967296);
    if s0 == 0, s0 = 1; end
    rngState = uint32(s0);
    for k = 1:8, rngState = local_xs32(rngState); end
end
z = zeros(1,6);
for k = 1:3
    rngState = local_xs32(rngState); u1 = double(rngState) / 4294967296;
    rngState = local_xs32(rngState); u2 = double(rngState) / 4294967296;
    r = sqrt(-2 * log(u1));
    z(2*k-1) = r * cos(2*pi*u2); z(2*k) = r * sin(2*pi*u2);
end
noise_I = 0.05 * z(1:3); noise_V = 0.50 * z(4:6);
I = [Ia, Ib, Ic] + noise_I; V = [Va, Vb, Vc] + noise_V;
bufI(:,idx) = I; bufV(:,idx) = V; idx = mod(idx, N) + 1;
Irms = sqrt(mean(bufI.^2, 2));
Crest = max(abs(bufI), [], 2) ./ max(Irms, 1e-6);
THD = zeros(3,1); Phase = zeros(3,1);
for p = 1:3
    Fi = fft(bufI(p,:)); Fv = fft(bufV(p,:));
    fundBin = round(50 * N / 1e4) + 1;
    fundMag = abs(Fi(fundBin)); harmMag = sqrt(sum(abs(Fi(fundBin+1:round(N/2))).^2));
    THD(p) = harmMag / max(fundMag, 1e-6);
    Phase(p) = angle(Fv(fundBin) * conj(Fi(fundBin)));   % V-I angle wrapped to (-pi, pi]
end
Irms_A=Irms(1); Irms_B=Irms(2); Irms_C=Irms(3);
Crest_A=Crest(1); Crest_B=Crest(2); Crest_C=Crest(3);
THD_A=THD(1); THD_B=THD(2); THD_C=THD(3);
Phase_A=Phase(1); Phase_B=Phase(2); Phase_C=Phase(3);
end
function x = local_xs32(x)
x = bitxor(x, bitshift(x, 13));
x = bitxor(x, bitshift(x, -17));
x = bitxor(x, bitshift(x, 5));
end

== matlab function fault_detection_system_v8/Sensing_ThreePhase/Fault_Injector ==
  data: VaIn input; Ia output; VbIn input; VcIn input; t input; FaultG input; FaultA input; FaultB input; FaultC input; MechanismCode input; Severity input; RampDuration input; FaultOnsetTime input; FaultDuration input; SourceL input; ReclosDelay input; BreakerOpen input; Ib output; Ic output; Va output; Vb output; Vc output; fault_flag output; G output; A output; B output; C output; reclose output
function [Ia,Ib,Ic,Va,Vb,Vc,fault_flag,G,A,B,C,reclose] = fault_injector(VaIn,VbIn,VcIn,t,FaultG,FaultA,FaultB,FaultC,MechanismCode,Severity,RampDuration,FaultOnsetTime,FaultDuration,SourceL,ReclosDelay,BreakerOpen)
%#codegen
persistent I_s I_src faultSamples initialized
if isempty(initialized)
    I_s = zeros(3,1); I_src = zeros(3,1); faultSamples = 0; initialized = true;
end
Ts = 1e-4; L = 0.02; R_normal = 5; R_source = 0.5;
% Source inductance as a backward-Euler equivalent resistance: Ls*(Iline[k]-Iline[k-1])/Ts = Vs - Rs*Iline[k] - Vt
Lr = SourceL / Ts; W = R_source + Lr;
fault_active = (t >= FaultOnsetTime) && (t < FaultOnsetTime + FaultDuration);
if fault_active, faultSamples = faultSamples + 1; else, faultSamples = 0; end
rampSamples = max(1, round(RampDuration / Ts)); frac = min(1, faultSamples / rampSamples);
flt = [double(FaultA); double(FaultB); double(FaultC)] > 0.5;
% 1. Source voltages and per-phase load resistance (mechanisms 3-6 act on one phase independently)
V_s = [VaIn; VbIn; VcIn];
R_load = [R_normal; R_normal; R_normal];
open_ph = false(3,1); R_open = R_normal;
if fault_active
    if MechanismCode == 3
        R_load(flt) = R_normal + frac * (Severity - R_normal);
    elseif MechanismCode == 4 || MechanismCode == 5
        V_s(flt) = V_s(flt) * (1 + frac * (Severity - 1));
    elseif MechanismCode == 6
        open_ph = flt; R_open = R_normal + frac * (Severity - R_normal);
    end
end
% 2. Fault admittance matrix at the terminal bus (short circuits only, mechanism 2)
%    LG / LLG / LLLG: Severity ohm from each faulted phase to ground
%    LL / LLL       : Severity ohm between each pair of faulted phases (cross-coupling terms)
Y_f = zeros(3,3);
if fault_active && MechanismCode == 2
    g_f = frac / max(Severity, 1e-6);
    if FaultG > 0.5
        for k = 1:3
            if flt(k), Y_f(k,k) = g_f; end
        end
    else
        for k = 1:3
            m = mod(k, 3) + 1;
            if flt(k) && flt(m)
                Y_f(k,k) = Y_f(k,k) + g_f; Y_f(m,m) = Y_f(m,m) + g_f;
                Y_f(k,m) = Y_f(k,m) - g_f; Y_f(m,k) = Y_f(m,k) - g_f;
            end
        end
    end
end
% 3. Terminal bus voltage. Load: I_new = c + a*Vt with c = I_s - a*R_load.*I_s and a = Ts/L.
%    Line (source side): W*I_line = Vs - Vt + Lr*I_src, with I_line = I_new + Y_f*Vt.
%    => ((1 + W*a)*I + W*Y_f) * Vt = Vs - W*c + Lr*I_src
a_l = Ts / L;
c_vec = I_s - a_l * (R_load .* I_s);
M = (1 + W * a_l) * eye(3) + W * Y_f;
V_t = M \ (V_s - W * c_vec + Lr * I_src);
I_new = c_vec + a_l * V_t;
% 4. Open-circuit phases: load current decays, bus voltage is the source voltage (as in v6)
for k = 1:3
    if open_ph(k)
        I_new(k) = I_s(k) * exp(-Ts * (R_open + R_source) / L);
        V_t(k) = V_s(k);
    end
end
% 5. Measured line current = load current + fault current (CT upstream of the fault, downstream of the breaker).
%    Breaker open: ideal interruption, every current is zero, the bus shows the source voltage.
if BreakerOpen > 0.5
    I_new = zeros(3,1); I_line = zeros(3,1); V_t = V_s;
else
    I_line = I_new + Y_f * V_t;
end
I_s = I_new; I_src = I_line;
Ia = I_line(1); Ib = I_line(2); Ic = I_line(3);
Va = V_t(1); Vb = V_t(2); Vc = V_t(3);
fault_flag = fault_active;
G = double(FaultG); A = double(FaultA); B = double(FaultB); C = double(FaultC);
tRec = FaultOnsetTime + FaultDuration + ReclosDelay;
reclose = double(t >= tRec && t < tRec + 1e-3);
end

== matlab function fault_detection_system_v8/Sequence_Components_3ph/Seq_3ph ==
  data: Ia input; I1 output; Ib input; Ic input; Va input; Vb input; Vc input; I2 output; I0 output; Unbal2 output; Unbal0 output; UnbalV0 output
function [I1,I2,I0,Unbal2,Unbal0,UnbalV0] = seq_3ph(Ia,Ib,Ic,Va,Vb,Vc)
%#codegen
persistent buf idx n cosW sinW wsum I1ref V1ref
N = 200; WARMUP = 500; USE_HANN = true;
LAM = 1e-3; NORMAL_UNBAL = 0.02; NORMAL_STEP = 0.02;
if isempty(idx)
    buf = zeros(6,N); idx = 1; n = 0; I1ref = 0; V1ref = 0;
    j = 0:N-1; w = ones(1,N);
    if USE_HANN, w = 0.5 * (1 - cos(2*pi*j/N)); end
    cosW = cos(2*pi*j/N) .* w; sinW = -sin(2*pi*j/N) .* w; wsum = sum(w);
end
buf(:,idx) = [Ia; Ib; Ic; Va; Vb; Vc]; idx = mod(idx, N) + 1; n = n + 1;
ord = mod((0:N-1) + idx - 1, N) + 1;
bo = buf(:, ord);
re = bo * cosW.'; im = bo * sinW.';
P = complex(re, im) * (sqrt(2) / wsum);
a = complex(-0.5, sqrt(3)/2); a2 = conj(a);
p1 = (P(1) + a*P(2) + a2*P(3)) / 3;
p2 = (P(1) + a2*P(2) + a*P(3)) / 3;
p0 = (P(1) + P(2) + P(3)) / 3;
v1 = (P(4) + a*P(5) + a2*P(6)) / 3;
v0 = (P(4) + P(5) + P(6)) / 3;
I1 = abs(p1); I2 = abs(p2); I0 = abs(p0); V1 = abs(v1);
if n <= WARMUP
    I1ref = I1; V1ref = V1;
else
    normalUnbal = (I2 / max(I1ref, 1e-6) < NORMAL_UNBAL) && (I0 / max(I1ref, 1e-6) < NORMAL_UNBAL);
    if normalUnbal && abs(I1 - I1ref) <= NORMAL_STEP * I1ref
        I1ref = I1ref + LAM * (I1 - I1ref);
    end
    if normalUnbal && abs(V1 - V1ref) <= NORMAL_STEP * V1ref
        V1ref = V1ref + LAM * (V1 - V1ref);
    end
end
Unbal2 = I2 / max(I1ref, 1e-6);
Unbal0 = I0 / max(I1ref, 1e-6);
UnbalV0 = abs(v0) / max(V1ref, 1e-6);
